simulink model "sschdlexThreePhaseConverterWithGridModel"  (R2026a)
settings: Solver=FixedStepDiscrete  StartTime=0  StopTime=0.09
InitFcn:
  | % LC filter parameters
  | 
  | Lf = 2e-3;
  | Rf = 20e-3;
  | Cf = 1e-6;
  | 
  | % Sample step size
  | 
  | % if ~exist('Tbase')
  |     Tbase = 5e-9;
  | % end
  | 
  | Ts = 1e-6;
  | Tsc=5e-5;
  | fsw = 10e3;
  | 
  | % PWM oversampling
  | oversampling = Ts/Tbase;
  | 
  | % Frame size for data transfer to CPU
  | frame_size = round(Tsc/Ts);
  | 
  | % Control constants
  | 
  | Kp_id = 1.5;
  | Ki_id = 400;
  | Kp_iq = 1.5;
  | Ki_iq = 400;
libraries: simulink x51, hdlsllib x23, fl_lib x15, nesl_utility x15, slrealtimeloglib x12, ee_lib x11, eeTransforms x3, slpidlib x2, eeSinusoidalMeasurement x1
(part 1 of 2)
settings Model: Creator=The MathWorks, Inc.  LastModifiedBy=The MathWorks, Inc.
settings OptimizationCC: ConditionallyExecuteInputs=off
settings DebuggingCC: AlgebraicLoopMsg=error  UnderspecifiedInitializationDetection=Classic  SingleTaskRateTransMsg=error  ParameterPrecisionLossMsg=none
settings HardwareCC: ProdHWDeviceType=ASIC/FPGA->ASIC/FPGA  TargetBitPerLong=64.0  TargetBitPerPointer=64.0  TargetBitPerSizeT=64.0  TargetBitPerPtrDiffT=64.0  TargetLongLongMode=on  TargetIntDivRoundTo=Zero  TargetEndianess=LittleEndian  TargetWordSize=64.0  TargetHWDeviceType=Custom Processor->MATLAB Host Computer  ProdEqTarget=off
settings GRTTargetCC: CombineOutputUpdateFcns=off  GRTInterface=on
settings SimscapeCC: SimscapeNormalizeSystem=off  SimscapeNominalValues="[{\"value\":\"1\",\"unit\":\"A\"},{\"value\":\"1\",\"unit\":\"bar\"},{\"value\":\"1\",\"unit\":\"cm^2\"},{\"value\":\"1\",\"unit\":\"cm^3/s\"},{\"value\":\"1\",\"unit\":\"kJ/kg\"},{\"value\":\"1\",\"unit\":\"kW\"},{\"value\":\"1\",\"unit\":\"l\"},{\"value\":\"1\",\"unit\":\"N\"},{\"value\":\"1\",\"unit\":\"N*m\"},{\"value\":\"1\",\"unit\":\"V\"}]"  SimscapeLogType=none  SimscapeLogDataHistory=5000.0

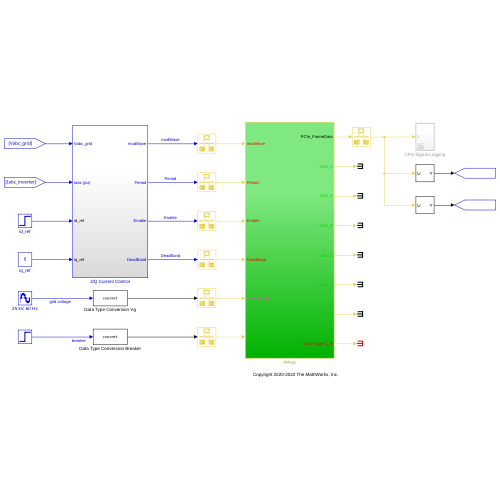
[thumbnail: Simulink's stored preview of the top-level diagram]
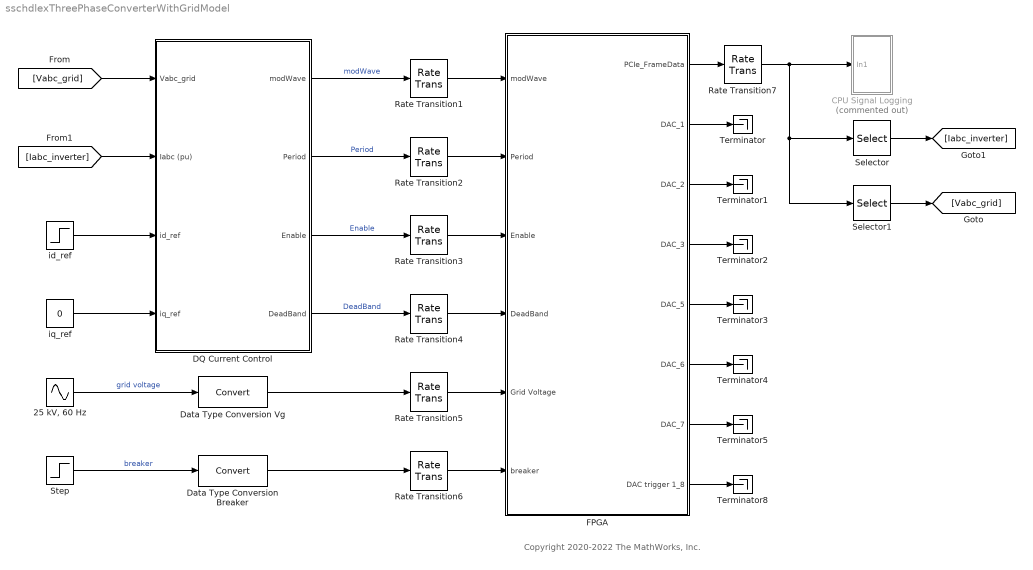
== system sschdlexThreePhaseConverterWithGridModel ==
  note: Copyright 2020-2022 The MathWorks, Inc.
  "25 kV, 60 Hz" : Sin  Amplitude=25000*sqrt(2)/sqrt(3)  Frequency=60*2*pi  Phase=[0 -2*pi/3 2*pi/3]  SampleTime=Tsc
  CPU Signal Logging : Subsystem  Commented=on
  DQ Current Control : Subsystem
  Data Type Conversion Breaker : DataTypeConversion  SaturateOnIntegerOverflow=off  RndMeth=Floor
  Data Type Conversion Vg : DataTypeConversion  SaturateOnIntegerOverflow=off  RndMeth=Floor
  FPGA : Subsystem
  Rate Transition{1..4} (4 alike) : RateTransition  OutPortSampleTime=Tbase
  Rate Transition5 : RateTransition  OutPortSampleTime=Ts
  Rate Transition6 : RateTransition  OutPortSampleTime=Ts
  Rate Transition7 : RateTransition  OutPortSampleTime=Tsc
  Selector : Selector  InputPortWidth=6*frame_size  IndexOptions=Index vector (dialog)  Indices=[1, frame_size+1, 2*frame_size+1]  OutputSizes=1
  Selector1 : Selector  InputPortWidth=6*frame_size  IndexOptions=Index vector (dialog)  Indices=[3*frame_size+1, 4*frame_size+1, 5*frame_size+1]  OutputSizes=1
  Step : Step  Time=0.03  SampleTime=Tsc
  Terminator{,1..5,8} (7 alike) : Terminator
  id_ref : Step  Time=0.06  FinalValue=0.5  SampleTime=Tsc
  iq_ref : Constant  Value=0  SampleTime=Tsc
  wires:
  DQ Current Control/1(modWave) -> Rate Transition1/1  "modWave"
  DQ Current Control/2(Period) -> Rate Transition2/1  "Period"
  DQ Current Control/4(DeadBand) -> Rate Transition4/1  "DeadBand"
  [Iabc_inverter] -> DQ Current Control/2(Iabc (pu))
  [Vabc_grid] -> DQ Current Control/1(Vabc_grid)
  DQ Current Control/3(Enable) -> Rate Transition3/1  "Enable"
  Step/1 -> Data Type Conversion Breaker/1  "breaker"
  FPGA/2(DAC_1) -> Terminator/1
  FPGA/3(DAC_2) -> Terminator1/1
  FPGA/4(DAC_3) -> Terminator2/1
  FPGA/5(DAC_5) -> Terminator3/1
  FPGA/6(DAC_6) -> Terminator4/1
  FPGA/7(DAC_7) -> Terminator5/1
  "25 kV, 60 Hz"/1 -> Data Type Conversion Vg/1  "grid voltage"
  FPGA/8(DAC trigger 1_8) -> Terminator8/1
  Rate Transition1/1 -> FPGA/1(modWave)
  Rate Transition2/1 -> FPGA/2(Period)
  Rate Transition3/1 -> FPGA/3(Enable)
  Rate Transition4/1 -> FPGA/4(DeadBand)
  Rate Transition5/1 -> FPGA/5(Grid Voltage)
  Rate Transition6/1 -> FPGA/6(breaker)
  FPGA/1(PCIe_FrameData) -> Rate Transition7/1
  id_ref/1 -> DQ Current Control/3(id_ref)
  iq_ref/1 -> DQ Current Control/4(iq_ref)
  Rate Transition7/1 -> Selector1/1, Selector/1, CPU Signal Logging/1(In1)
  Data Type Conversion Vg/1 -> Rate Transition5/1
  Data Type Conversion Breaker/1 -> Rate Transition6/1
  Selector/1 -> [Iabc_inverter]
  Selector1/1 -> [Vabc_grid]

== system sschdlexThreePhaseConverterWithGridModel/CPU Signal Logging ==
  In1 : Inport
  Demux : Demux  Outputs=12
  File Log{,1..11} (12 alike) : slrealtimeloglib/File Log  decimation=1
  wires:
  Demux/3 -> File Log2/1
  Demux/2 -> File Log1/1
  Demux/1 -> File Log/1
  In1/1 -> Demux/1
  Demux/5 -> File Log4/1
  Demux/12 -> File Log11/1
  Demux/4 -> File Log3/1
  Demux/9 -> File Log8/1
  Demux/6 -> File Log5/1
  Demux/10 -> File Log9/1
  Demux/11 -> File Log10/1
  Demux/8 -> File Log7/1
  Demux/7 -> File Log6/1

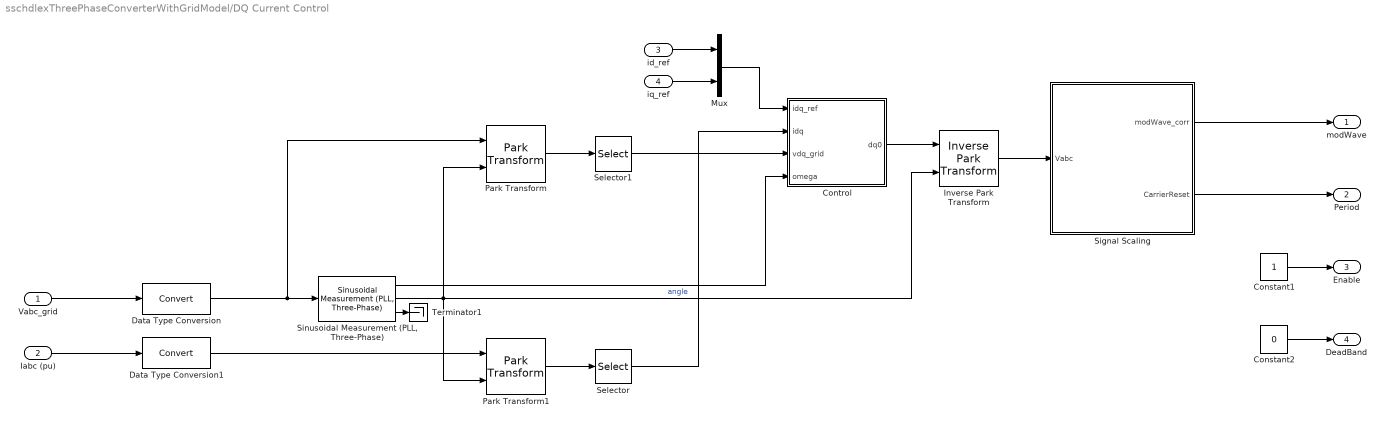
== system sschdlexThreePhaseConverterWithGridModel/DQ Current Control ==
  Vabc_grid : Inport
  Iabc (pu) : Inport  Port=2
  id_ref : Inport  Port=3
  iq_ref : Inport  Port=4
  Constant1 : Constant  OutDataTypeStr=boolean  SampleTime=Tsc
  Constant2 : Constant  Value=0  OutDataTypeStr=uint32  SampleTime=Tsc
  Control : Subsystem
  Data Type Conversion : DataTypeConversion  SaturateOnIntegerOverflow=off  RndMeth=Floor
  Data Type Conversion1 : DataTypeConversion  SaturateOnIntegerOverflow=off  RndMeth=Floor
  Inverse Park Transform : eeTransforms/Inverse Park Transform  AxisAlignment=Q-axis  PowerInvariant=off
  Mux : Mux  Inputs=2
  Park Transform : eeTransforms/Park Transform  AxisAlignment=Q-axis  PowerInvariant=off
  Park Transform1 : eeTransforms/Park Transform  AxisAlignment=Q-axis  PowerInvariant=off
  Selector : Selector  InputPortWidth=3  IndexOptions=Index vector (dialog)  Indices=[1 2]  OutputSizes=1
  Selector1 : Selector  InputPortWidth=3  IndexOptions=Index vector (dialog)  Indices=[1 2]  OutputSizes=1
  Signal Scaling : Subsystem  mask{Vdc=2, fsw=20e3, f_FPGA_clk=1/Tbase}
      mask prompts: fsw "PWM Frequency"; f_FPGA_clk "FPGA Target Frequency"
  "Sinusoidal Measurement (PLL, Three-Phase)" : eeSinusoidalMeasurement/Sinusoidal Measurement (PLL, Three-Phase)  Kp_LF=150  Ki_LF=150  F0=60  Theta0=0  Ts=Tsc
  Terminator1 : Terminator
  modWave : Outport
  Period : Outport  Port=2
  Enable : Outport  Port=3
  DeadBand : Outport  Port=4
  wires:
  Constant1/1 -> Enable/1
  Signal Scaling/1(modWave_corr) -> modWave/1
  Signal Scaling/2(CarrierReset) -> Period/1
  Constant2/1 -> DeadBand/1
  Inverse Park Transform/1 -> Signal Scaling/1(Vabc)
  Mux/1 -> Control/1(idq_ref)
  id_ref/1 -> Mux/1
  iq_ref/1 -> Mux/2
  Selector1/1 -> Control/3(vdq_grid)
  Data Type Conversion/1 -> "Sinusoidal Measurement (PLL, Three-Phase)"/1, Park Transform/1
  "Sinusoidal Measurement (PLL, Three-Phase)"/2 -> Park Transform/2, Inverse Park Transform/2, Park Transform1/2  "angle"
  Control/1(dq0) -> Inverse Park Transform/1
  Park Transform/1 -> Selector1/1
  "Sinusoidal Measurement (PLL, Three-Phase)"/1 -> Control/4(omega)
  Park Transform1/1 -> Selector/1
  Selector/1 -> Control/2(idq)
  "Sinusoidal Measurement (PLL, Three-Phase)"/3 -> Terminator1/1
  Data Type Conversion1/1 -> Park Transform1/1
  Vabc_grid/1 -> Data Type Conversion/1
  Iabc (pu)/1 -> Data Type Conversion1/1

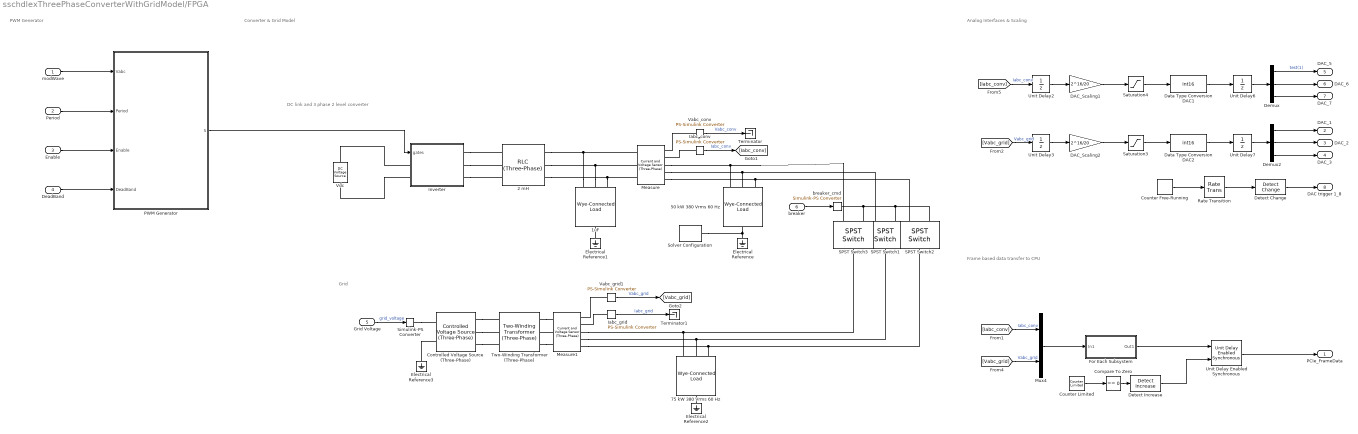
== system sschdlexThreePhaseConverterWithGridModel/FPGA ==
  note: Frame based data transfer to CPU
  note: Analog Interfaces & Scaling
  note: Converter & Grid Model
  note: PWM Generator
  note: Grid
  note: DC link and 3 phase 2 level converter
  modWave : Inport
  Period : Inport  Port=2
  Enable : Inport  Port=3
  DeadBand : Inport  Port=4
  Grid Voltage : Inport  Port=5
  breaker : Inport  Port=6
  1uF : ee_lib/Passive/RLC Assemblies/Wye-Connected Load  port_option=ee.enum.threePhasePort.expanded  parameterization=1  component_structure=3  component_structure_PQ=3  R=1 Ohm  L=0.001 H  C=Cf F  VRated=380 V  FRated=60 Hz  P=0 W  Qpos=0 V*A  Qneg="-54.4375  V*A"  R_parasitic=1e-6 Ohm  G_parasitic=1e-6 1/Ohm  R_parasitic_PQ=1e-6 Ohm  G_parasitic_PQ=1e-6 1/Ohm  Vmag0=380 V  Vang0=0 deg  Freq0=60 Hz  IL_specify=on  IL_priority=High  IL=[ 0 0 0 ] A  IL_nominal_specify=off  IL_nominal_value=1  IL_nominal_unit=A  VC_specify=on  VC_priority=High  VC=[ 0 0 0 ] V  VC_nominal_specify=off  VC_nominal_value=1  VC_nominal_unit=V
  "2 mH " : ee_lib/Passive/RLC Assemblies/RLC (Three-Phase)  port_option=ee.enum.threePhasePort.expanded  component_structure=ee.enum.rlc.structure.SeriesRL  R=Rf Ohm  L=Lf H  C=1 F  R_parasitic=1e-6 Ohm  G_parasitic=1e-6 1/Ohm  IL_specify=on  IL_priority=High  IL=[0, 0, 0] A  IL_nominal_specify=off  IL_nominal_value=1  IL_nominal_unit=A  VC_specify=on  VC_priority=High  VC=[0, 0, 0] V  VC_nominal_specify=off  VC_nominal_value=1  VC_nominal_unit=V
  50 kW 380 Vrms 60 Hz : ee_lib/Passive/RLC Assemblies/Wye-Connected Load  port_option=ee.enum.threePhasePort.expanded  parameterization=2  component_structure=3  component_structure_PQ=1  R=1 Ohm  L=0.001 H  C=1e-6 F  VRated=380 V  FRated=60 Hz  P=50000 W  Qpos=0 V*A  Qneg=-3000 V*A  R_parasitic=1e-6 Ohm  G_parasitic=1e-6 1/Ohm  R_parasitic_PQ=1e-6 Ohm  G_parasitic_PQ=1e-6 1/Ohm  Vmag0=380 V  Vang0=0 deg  Freq0=60 Hz  IL_specify=on  IL_priority=High  IL=[ 0 0 0 ] A  IL_nominal_specify=off  IL_nominal_value=1  IL_nominal_unit=A  VC_specify=on  VC_priority=High  VC=[ 0 0 0 ] V  VC_nominal_specify=off  VC_nominal_value=1  VC_nominal_unit=V
  75 kW 380 Vrms 60 Hz : ee_lib/Passive/RLC Assemblies/Wye-Connected Load  port_option=ee.enum.threePhasePort.expanded  parameterization=2  component_structure=3  component_structure_PQ=1  R=1 Ohm  L=0.001 H  C=1e-6 F  VRated=380 V  FRated=60 Hz  P=75000 W  Qpos=0 V*A  Qneg=-3000 V*A  R_parasitic=1e-6 Ohm  G_parasitic=1e-6 1/Ohm  R_parasitic_PQ=1e-6 Ohm  G_parasitic_PQ=1e-6 1/Ohm  Vmag0=380 V  Vang0=0 deg  Freq0=60 Hz  IL_specify=on  IL_priority=High  IL=[ 0 0 0 ] A  IL_nominal_specify=off  IL_nominal_value=1  IL_nominal_unit=A  VC_specify=on  VC_priority=High  VC=[ 0 0 0 ] V  VC_nominal_specify=off  VC_nominal_value=1  VC_nominal_unit=V
  Compare To Zero : simulink/Logic and Bit Operations/Compare To Zero  relop===  OutDataTypeStr=boolean
  Controlled Voltage Source (Three-Phase) : ee_lib/Sources/Controlled Voltage Source (Three-Phase)  input_option=ee.enum.inputType.instantaneous  FRated=60 Hz
  Counter Free-Running : simulink/Sources/Counter Free-Running  NumBits=1  tsamp=Ts
  Counter Limited : simulink/Sources/Counter Limited  uplimit=frame_size-1  tsamp=Ts
  DAC_Scaling1 : Gain  Gain=2^16/20
  DAC_Scaling2 : Gain  Gain=2^16/20
  Data Type Conversion DAC1 : DataTypeConversion  OutDataTypeStr=int16  SaturateOnIntegerOverflow=off  RndMeth=Floor
  Data Type Conversion DAC2 : DataTypeConversion  OutDataTypeStr=int16  SaturateOnIntegerOverflow=off  RndMeth=Floor
  Demux : Demux  Outputs=3
  Demux2 : Demux  Outputs=3
  Detect Change : simulink/Logic and Bit Operations/Detect Change  vinit=0  OutDataTypeStr=boolean
  Detect Increase : simulink/Logic and Bit Operations/Detect Increase  vinit=0.0  OutDataTypeStr=boolean
  Electrical Reference{,1..3} (4 alike) : fl_lib/Electrical/Electrical Elements/Electrical Reference
  For Each Subsystem : Subsystem  TreatAsAtomicUnit=on
  Iabc_conv : nesl_utility/PS-Simulink Converter  PhysicalDomain=network_engine_domain  SubClassName=ps_output  LeftPortType=input  RightPortType=output  PseudoPeriodic=off  Frequencies=[]  VectorFormat=1-D array  Unit=inherit  AffineConversion=off
  Iabc_grid : nesl_utility/PS-Simulink Converter  PhysicalDomain=network_engine_domain  SubClassName=ps_output  LeftPortType=input  RightPortType=output  PseudoPeriodic=off  Frequencies=[]  VectorFormat=1-D array  Unit=inherit  AffineConversion=off
  Inverter : Subsystem
      mask Display: %image('Inverter.png'); % Use "Edit Image" on toolstrip to change.
  Measure : ee_lib/Sensors & Transducers/Current and Voltage Sensor (Three-Phase)  port_option=ee.enum.threePhasePort.expanded  vMeasurementType=ee.enum.vmeasurement.lg  outputUnit=ee.enum.unit.pu  SRated=150000 V*A  VRated=380 V  I_specify=off  I_priority=None  I=[ 0 0 0 ] A  I_nominal_specify=off  I_nominal_value=1  I_nominal_unit=A  V_specify=off  V_priority=None  V=[ 0 0 0 ] V  V_nominal_specify=off  V_nominal_value=1  V_nominal_unit=V
  Measure1 : ee_lib/Sensors & Transducers/Current and Voltage Sensor (Three-Phase)  port_option=ee.enum.threePhasePort.expanded  vMeasurementType=ee.enum.vmeasurement.lg  outputUnit=ee.enum.unit.pu  SRated=250000 V*A  VRated=380 V  I_specify=off  I_priority=None  I=[ 0 0 0 ] A  I_nominal_specify=off  I_nominal_value=1  I_nominal_unit=A  V_specify=off  V_priority=None  V=[ 0 0 0 ] V  V_nominal_specify=off  V_nominal_value=1  V_nominal_unit=V
  Mux4 : Mux  Inputs=2
  PWM Generator : Subsystem
  Rate Transition : RateTransition  OutPortSampleTime=Tbase
  SPST Switch1 : ee_lib/Switches & Breakers/SPST Switch  R_closed=0.001 Ohm  G_open=1e-6 S  Threshold=0.5 V  Width=0 V  model_dynamics=0  t_on=1e-3 s  t_off=1e-3 s  initial_vT=0 V
  SPST Switch2 : ee_lib/Switches & Breakers/SPST Switch  R_closed=0.001 Ohm  G_open=1e-6 S  Threshold=0.5 V  Width=0 V  model_dynamics=0  t_on=1e-3 s  t_off=1e-3 s  initial_vT=0 V
  SPST Switch3 : ee_lib/Switches & Breakers/SPST Switch  R_closed=0.001 Ohm  G_open=1e-6 S  Threshold=0.5 V  Width=0 V  model_dynamics=0  t_on=1e-3 s  t_off=1e-3 s  initial_vT=0 V
  Saturation3 : Saturate  UpperLimit=2^15-1  LowerLimit=-2^15
  Saturation4 : Saturate  UpperLimit=2^15-1  LowerLimit=-2^15
  Simulink-PS Converter : nesl_utility/Simulink-PS Converter  PhysicalDomain=network_engine_domain  SubClassName=ps_input  LeftPortType=input  RightPortType=output  PseudoPeriodic=off  Frequencies=[]  NoiseDistribution=none  NoiseParameters=[]  Unit=1  AffineConversion=off  FilteringAndDerivatives=provide  SimscapeFilterOrder=1  InputFilterTimeConstant=0.001  UdotUserProvided=0
  Solver Configuration : nesl_utility/Solver Configuration  PhysicalDomain=network_engine_domain  SubClassName=solver  LeftPortType=input  RightPortType=generic  Tones=[]  Harmonics=[]  SimulateNoise=off  Profile=off  UseLocalSampling=off  EnableSwitchedLinearOptims=on  FrequencyDomain=off  UseCCode=off  RelTol=0.001  AbsTol=1e-06  MinStep=1e-09  ToWorkspace=off  RevertToSquareIcSolve=off  NumHomotopyIterations=100  PhasorMode=off  PhasorModeNumHarmonics=1  ConsistencySolver=NEWTON_FTOL  CanonicalOrdering=UNORDERED  OptimizeIntermediates=UNOPTIMIZED  IndexReductionMethod=DerivativeReplacement  DoDC=off  ResidualTolerance=1e-09  ConsistencyTolSource=GLOBAL  ConsistencyAbsTol=0.001  ConsistencyRelTol=0.001  ConsistencyTolFactor=0.001  UseLocalSolver=on  LocalSolverChoice=NE_BACKWARD_EULER_ADVANCER  ResolveIndetEquations=on  FunctionEvalNumThread=1  LocalSolverSampleTime=Ts  DoFixedCost=on  MaxNonlinIter=1  MaxModeIter=2  ComputeImpulses=off  ImpulseIterations=1  LinearAlgebra=Sparse  LinearAlgebraNumThread=0  EquationFormulation=NE_TIME_EF  DelaysMemoryBudget=1024  AutomaticFiltering=on  FilteringTimeConstant=0.001  PartitionStorageMethod=EXHAUSTIVE  PartitionMemoryBudget=1024  PartitionMethod=ROBUST  MultibodyUseLocalSolver=off  MultibodyLocalSolverChoice=ODE1  MultibodyLocalSolverSampleTime=0.001
  Terminator : Terminator
  Terminator1 : Terminator
  Two-Winding Transformer (Three-Phase) : ee_lib/Passive/Transformers/Two-Winding Transformer (Three-Phase)  SRated=500000 V*A  FRated=60 Hz  Winding1Connection=ee.enum.windingconnection.Y  VRated1=25000 V  Winding2Connection=ee.enum.windingconnection.delta1  VRated2=380 V  CoreType=ee.enum.coretype.threelimb  pu_Rw1=0.0020  pu_Rw2=0.0020  leakage_reactance_option=ee.enum.transformer_leakage.include  pu_Xl1=0.0800  pu_Xl2=0.0800  magnetizing_resistance_option=ee.enum.transformer_magnetizingResistance.include  pu_Rm=500  magnetizing_reactance_option=ee.enum.transformer_magnetizingReactance.include  saturation_option=ee.enum.transformer_saturation.exclude  pu_Xm=500  current_data=[0, .002, 1, 2]  magnetic_flux_data=[0, 1.2, 1.5, 1.51]  pu_X0=0.5800  i1_specify=off  i1_priority=None  i1=[ 0 0 0 ] A  i1_nominal_specify=off  i1_nominal_value=1  i1_nominal_unit=A  i2_specify=off  i2_priority=None  i2=[ 0 0 0 ] A  i2_nominal_specify=off  i2_nominal_value=1  i2_nominal_unit=A  phi_specify=off  phi_priority=None  phi=[ 0 0 0 ]  phi_nominal_specify=off  phi_nominal_value=1  phi_nominal_unit=1
  Unit Delay Enabled Synchronous : hdlsllib/Discrete/Unit Delay Enabled Synchronous  InitialCondition=0.0  SampleTime=-1
  Unit Delay{2..3,6..7} (4 alike) : UnitDelay  SampleTime=-1
  Vabc_conv : nesl_utility/PS-Simulink Converter  PhysicalDomain=network_engine_domain  SubClassName=ps_output  LeftPortType=input  RightPortType=output  PseudoPeriodic=off  Frequencies=[]  VectorFormat=1-D array  Unit=inherit  AffineConversion=off
  Vabc_grid1 : nesl_utility/PS-Simulink Converter  PhysicalDomain=network_engine_domain  SubClassName=ps_output  LeftPortType=input  RightPortType=output  PseudoPeriodic=off  Frequencies=[]  VectorFormat=1-D array  Unit=inherit  AffineConversion=off
  Vdc : fl_lib/Electrical/Electrical Sources/DC Voltage Source  v0=1000 V
  breaker_cmd : nesl_utility/Simulink-PS Converter  PhysicalDomain=network_engine_domain  SubClassName=ps_input  LeftPortType=input  RightPortType=output  PseudoPeriodic=off  Frequencies=[]  NoiseDistribution=none  NoiseParameters=[]  Unit=1  AffineConversion=off  FilteringAndDerivatives=provide  SimscapeFilterOrder=1  InputFilterTimeConstant=0.001  UdotUserProvided=0
  PCIe_FrameData : Outport
  DAC_1 : Outport  Port=2
  DAC_2 : Outport  Port=3
  DAC_3 : Outport  Port=4
  DAC_5 : Outport  Port=5
  DAC_6 : Outport  Port=6
  DAC_7 : Outport  Port=7
  DAC trigger 1_8 : Outport  Port=8
  wires:
  DeadBand/1 -> PWM Generator/4(DeadBand)
  modWave/1 -> PWM Generator/1(Vabc)
  Enable/1 -> PWM Generator/3(Enable)
  Period/1 -> PWM Generator/2(Period)
  Counter Free-Running/1 -> Rate Transition/1
  Rate Transition/1 -> Detect Change/1
  Demux/1 -> DAC_5/1  "test(1)"
  Demux/2 -> DAC_6/1
  Demux/3 -> DAC_7/1
  Demux2/1 -> DAC_1/1
  Demux2/2 -> DAC_2/1
  Demux2/3 -> DAC_3/1
  Unit Delay2/1 -> DAC_Scaling1/1
  Unit Delay3/1 -> DAC_Scaling2/1
  DAC_Scaling1/1 -> Saturation4/1
  DAC_Scaling2/1 -> Saturation3/1
  Saturation4/1 -> Data Type Conversion DAC1/1
  Saturation3/1 -> Data Type Conversion DAC2/1
  Unit Delay6/1 -> Demux/1
  Unit Delay7/1 -> Demux2/1
  Data Type Conversion DAC1/1 -> Unit Delay6/1
  Data Type Conversion DAC2/1 -> Unit Delay7/1
  Detect Change/1 -> DAC trigger 1_8/1
  Mux4/1 -> For Each Subsystem/1(In1)
  Iabc_conv/1 -> [Iabc_conv]  "Iabc_conv"
  Vabc_conv/1 -> Terminator/1  "Vabc_conv"
  Vabc_grid1/1 -> [Vabc_grid]  "Vabc_grid"
  Iabc_grid/1 -> Terminator1/1  "Iabc_grid"
  PWM Generator/1(S) -> Inverter/1(gates)
  Grid Voltage/1 -> Simulink-PS Converter/1  "grid_voltage"
  breaker/1 -> breaker_cmd/1
  [Vabc_grid] -> Unit Delay3/1  "Vabc_grid"
  [Iabc_conv] -> Unit Delay2/1  "Iabc_conv"
  [Vabc_grid] -> Mux4/2  "Vabc_grid"
  [Iabc_conv] -> Mux4/1  "Iabc_conv"
  Counter Limited/1 -> Compare To Zero/1
  Compare To Zero/1 -> Detect Increase/1
  Detect Increase/1 -> Unit Delay Enabled Synchronous/2
  Unit Delay Enabled Synchronous/1 -> PCIe_FrameData/1
  For Each Subsystem/1(Out1) -> Unit Delay Enabled Synchronous/1
  connections:
  SPST Switch1/LConn1 -- SPST Switch2/LConn1 -- SPST Switch3/LConn1 -- breaker_cmd/RConn1
  50 kW 380 Vrms 60 Hz/RConn1 -- Electrical Reference/LConn1 -- Solver Configuration/RConn1
  SPST Switch3/RConn1 -- 75 kW 380 Vrms 60 Hz/LConn1 -- Measure1/RConn3
  SPST Switch2/LConn2 -- 50 kW 380 Vrms 60 Hz/LConn3 -- Measure/RConn5
  50 kW 380 Vrms 60 Hz/LConn1 -- SPST Switch3/LConn2 -- Measure/RConn3
  1uF/LConn1 -- Measure/LConn1 -- "2 mH "/RConn1
  SPST Switch2/RConn1 -- 75 kW 380 Vrms 60 Hz/LConn3 -- Measure1/RConn5
  1uF/LConn3 -- Measure/LConn3 -- "2 mH "/RConn3
  SPST Switch1/LConn2 -- 50 kW 380 Vrms 60 Hz/LConn2 -- Measure/RConn4
  1uF/LConn2 -- Measure/LConn2 -- "2 mH "/RConn2
  SPST Switch1/RConn1 -- 75 kW 380 Vrms 60 Hz/LConn2 -- Measure1/RConn4
  Electrical Reference3/LConn1 -- Controlled Voltage Source (Three-Phase)/LConn2
  Inverter/RConn3 -- "2 mH "/LConn3
  Controlled Voltage Source (Three-Phase)/RConn3 -- Two-Winding Transformer (Three-Phase)/LConn3
  Controlled Voltage Source (Three-Phase)/RConn1 -- Two-Winding Transformer (Three-Phase)/LConn1
  Measure1/LConn2 -- Two-Winding Transformer (Three-Phase)/RConn2
  Iabc_conv/LConn1 -- Measure/RConn2
  Iabc_grid/LConn1 -- Measure1/RConn2
  Inverter/LConn1 -- Vdc/LConn1
  Inverter/RConn2 -- "2 mH "/LConn2
  Simulink-PS Converter/RConn1 -- Controlled Voltage Source (Three-Phase)/LConn1
  Two-Winding Transformer (Three-Phase)/RConn3 -- Measure1/LConn3
  Vabc_conv/LConn1 -- Measure/RConn1
  Electrical Reference2/LConn1 -- 75 kW 380 Vrms 60 Hz/RConn1
  Controlled Voltage Source (Three-Phase)/RConn2 -- Two-Winding Transformer (Three-Phase)/LConn2
  Two-Winding Transformer (Three-Phase)/RConn1 -- Measure1/LConn1
  Inverter/RConn1 -- "2 mH "/LConn1
  Vabc_grid1/LConn1 -- Measure1/RConn1
  Inverter/LConn2 -- Vdc/RConn1
  Electrical Reference1/LConn1 -- 1uF/RConn1

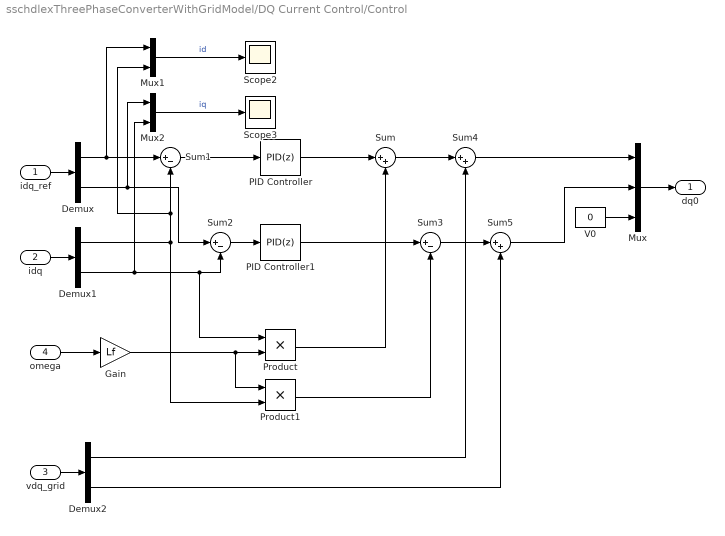
== system sschdlexThreePhaseConverterWithGridModel/DQ Current Control/Control ==
  idq_ref : Inport
  idq : Inport  Port=2
  vdq_grid : Inport  Port=3
  omega : Inport  Port=4
  Demux : Demux  Outputs=2
  Demux1 : Demux  Outputs=2
  Demux2 : Demux  Outputs=2
  Gain : Gain  Gain=Lf
  Mux : Mux  Inputs=3
  Mux1 : Mux  Inputs=2
  Mux2 : Mux  Inputs=2
  PID Controller : slpidlib/PID Controller  Controller=PID  Form=Parallel  TimeDomain=Discrete-time  UseExternalTs=off  SampleTime=-1  IntegratorMethod=Forward Euler  FilterMethod=Forward Euler  ControllerParametersSource=internal  P=Kp_id  I=Ki_id  UseKiTs=off  D=0  UseExternalDerivativeSource=off  N=100  UseFilter=off  TunerSelectOption=Transfer Function Based (PID Tuner App)  InitialConditionSource=internal  InitialConditionForIntegrator=0  InitialConditionForFilter=0  DifferentiatorICPrevScaledInput=0  ExternalReset=none  TrackingMode=off  Kt=1  LimitOutput=on  SatLimitsSource=internal  UpperSaturationLimit=3  LowerSaturationLimit=-3  LinearizeAsGain=on  AntiWindupMode=back-calculation  Kb=100  LimitIntegrator=off  UpperIntegratorSaturationLimit=inf  LowerIntegratorSaturationLimit=-inf  POutMin=[]  POutMax=[]  IOutMin=[]  IOutMax=[]  DOutMin=[]  DOutMax=[]  NOutMin=[]  NOutMax=[]  SumOutMin=[]  SumOutMax=[]  SaturationOutMin=[]  SaturationOutMax=[]  PParamMin=[]  PParamMax=[]  IParamMin=[]  IParamMax=[]  DParamMin=[]  DParamMax=[]  NParamMin=[]  NParamMax=[]  KbParamMin=[]  KbParamMax=[]  KtParamMin=[]  KtParamMax=[]  KbOutMin=[]  KbOutMax=[]  KtOutMin=[]  KtOutMax=[]  IntegratorOutMin=[]  IntegratorOutMax=[]  FilterOutMin=[]  FilterOutMax=[]  SumI1OutMin=[]  SumI1OutMax=[]  SumI2OutMin=[]  SumI2OutMax=[]  SumI3OutMin=[]  SumI3OutMax=[]  SumI4OutMin=[]  SumI4OutMax=[]  SumDOutMin=[]  SumDOutMax=[]  DifferentiatorOutMin=[]  DifferentiatorOutMax=[]  FilterDiffOutCoefMin=[]  FilterDiffOutCoefMax=[]  ReciprocalOutMin=[]  ReciprocalOutMax=[]  SumDenOutMin=[]  SumDenOutMax=[]  SumNumOutMin=[]  SumNumOutMax=[]  DivideOutMin=[]  DivideOutMax=[]  UdiffTsProdOutMin=[]  UdiffTsProdOutMax=[]  NTsProdOutMin=[]  NTsProdOutMax=[]  UintegralTsProdOutMin=[]  UintegralTsProdOutMax=[]  UngainTsProdOutMin=[]  UngainTsProdOutMax=[]  ClampingZeroOutDataTypeStr=Inherit: Inherit via back propagation  ClampingZeroOutMin=[]  ClampingZeroOutMax=[]  FilterDenConstantOutDataTypeStr=Inherit: Inherit via back propagation  FilterDenConstantOutMin=[]  FilterDenConstantOutMax=[]  PCopyOutDataTypeStr=Inherit: Inherit via back propagation  PCopyOutMin=[]  PCopyOutMax=[]  NCopyOutDataTypeStr=Inherit: Inherit via back propagation  NCopyOutMin=[]  NCopyOutMax=[]  IntegratorContinuousStateAttributes=''  IntegratorStateMustResolveToSignalObject=off  IntegratorRTWStateStorageClass=Auto  FilterContinuousStateAttributes=''  FilterStateMustResolveToSignalObject=off  FilterRTWStateStorageClass=Auto  ParallelPVariant=InternalParameters  IdealPVariant=Disabled  IVariant=InternalParameters  DVariant=InternalParameters  IntegratorVariant=Discrete  SatVariant=Enabled  AWVariant=BackCalculation  PCopyVariant=Disabled  TRVariant=Disabled  FdbkBlocksVariant=Forward  IdealPFdbkVariant=Disabled  SatFdbkVariant=Disabled  DerivativeFilterVariant=Differentiator  NVariant=Passthrough  NCopyVariant=Disabled_SignalSpec  FilterICVariant=InternalICsDifferentiator  IntegratorICVariant=InternalICs  ExternalResetVariant=Disabled  TRSumVariant=Passthrough  SumFdbkVariant=Disabled  SumVariant=Sum_PID  TsampFilterVariant=InternalTs  TsampNgainVariant=Passthrough  TsampIntegralVariant=Disabled_SignalSpec  ExternalSaturationOutDataTypeStr=Inherit: Same as second input  DerivativeSourceVariant=ErrorSignal  PreIntVariant=InternalPreInt
  PID Controller1 : slpidlib/PID Controller  Controller=PID  Form=Parallel  TimeDomain=Discrete-time  UseExternalTs=off  SampleTime=-1  IntegratorMethod=Forward Euler  FilterMethod=Forward Euler  ControllerParametersSource=internal  P=Kp_iq  I=Ki_iq  UseKiTs=off  D=0  UseExternalDerivativeSource=off  N=100  UseFilter=off  TunerSelectOption=Transfer Function Based (PID Tuner App)  InitialConditionSource=internal  InitialConditionForIntegrator=0  InitialConditionForFilter=0  DifferentiatorICPrevScaledInput=0  ExternalReset=none  TrackingMode=off  Kt=1  LimitOutput=on  SatLimitsSource=internal  UpperSaturationLimit=3  LowerSaturationLimit=-3  LinearizeAsGain=on  AntiWindupMode=back-calculation  Kb=100  LimitIntegrator=off  UpperIntegratorSaturationLimit=inf  LowerIntegratorSaturationLimit=-inf  POutMin=[]  POutMax=[]  IOutMin=[]  IOutMax=[]  DOutMin=[]  DOutMax=[]  NOutMin=[]  NOutMax=[]  SumOutMin=[]  SumOutMax=[]  SaturationOutMin=[]  SaturationOutMax=[]  PParamMin=[]  PParamMax=[]  IParamMin=[]  IParamMax=[]  DParamMin=[]  DParamMax=[]  NParamMin=[]  NParamMax=[]  KbParamMin=[]  KbParamMax=[]  KtParamMin=[]  KtParamMax=[]  KbOutMin=[]  KbOutMax=[]  KtOutMin=[]  KtOutMax=[]  IntegratorOutMin=[]  IntegratorOutMax=[]  FilterOutMin=[]  FilterOutMax=[]  SumI1OutMin=[]  SumI1OutMax=[]  SumI2OutMin=[]  SumI2OutMax=[]  SumI3OutMin=[]  SumI3OutMax=[]  SumI4OutMin=[]  SumI4OutMax=[]  SumDOutMin=[]  SumDOutMax=[]  DifferentiatorOutMin=[]  DifferentiatorOutMax=[]  FilterDiffOutCoefMin=[]  FilterDiffOutCoefMax=[]  ReciprocalOutMin=[]  ReciprocalOutMax=[]  SumDenOutMin=[]  SumDenOutMax=[]  SumNumOutMin=[]  SumNumOutMax=[]  DivideOutMin=[]  DivideOutMax=[]  UdiffTsProdOutMin=[]  UdiffTsProdOutMax=[]  NTsProdOutMin=[]  NTsProdOutMax=[]  UintegralTsProdOutMin=[]  UintegralTsProdOutMax=[]  UngainTsProdOutMin=[]  UngainTsProdOutMax=[]  ClampingZeroOutDataTypeStr=Inherit: Inherit via back propagation  ClampingZeroOutMin=[]  ClampingZeroOutMax=[]  FilterDenConstantOutDataTypeStr=Inherit: Inherit via back propagation  FilterDenConstantOutMin=[]  FilterDenConstantOutMax=[]  PCopyOutDataTypeStr=Inherit: Inherit via back propagation  PCopyOutMin=[]  PCopyOutMax=[]  NCopyOutDataTypeStr=Inherit: Inherit via back propagation  NCopyOutMin=[]  NCopyOutMax=[]  IntegratorContinuousStateAttributes=''  IntegratorStateMustResolveToSignalObject=off  IntegratorRTWStateStorageClass=Auto  FilterContinuousStateAttributes=''  FilterStateMustResolveToSignalObject=off  FilterRTWStateStorageClass=Auto  ParallelPVariant=InternalParameters  IdealPVariant=Disabled  IVariant=InternalParameters  DVariant=InternalParameters  IntegratorVariant=Discrete  SatVariant=Enabled  AWVariant=BackCalculation  PCopyVariant=Disabled  TRVariant=Disabled  FdbkBlocksVariant=Forward  IdealPFdbkVariant=Disabled  SatFdbkVariant=Disabled  DerivativeFilterVariant=Differentiator  NVariant=Passthrough  NCopyVariant=Disabled_SignalSpec  FilterICVariant=InternalICsDifferentiator  IntegratorICVariant=InternalICs  ExternalResetVariant=Disabled  TRSumVariant=Passthrough  SumFdbkVariant=Disabled  SumVariant=Sum_PID  TsampFilterVariant=InternalTs  TsampNgainVariant=Passthrough  TsampIntegralVariant=Disabled_SignalSpec  ExternalSaturationOutDataTypeStr=Inherit: Same as second input  DerivativeSourceVariant=ErrorSignal  PreIntVariant=InternalPreInt
  Product : Product
  Product1 : Product
  Scope2 : Scope
      settings: ActiveDisplayYMinimum=-1.23441  ActiveDisplayYMaximum=0.69271  DataLoggingVariableName=id
  Scope3 : Scope
      settings: ActiveDisplayYMinimum=-0.35108  ActiveDisplayYMaximum=0.28909  DataLoggingVariableName=iq
  Sum : Sum  Inputs=|++
  Sum1 : Sum  Inputs=|+-
  Sum2 : Sum  Inputs=|+-
  Sum3 : Sum  Inputs=|+-
  Sum4 : Sum  Inputs=|++
  Sum5 : Sum  Inputs=|++
  V0 : Constant  Value=0  SampleTime=-1
  dq0 : Outport
  wires:
  Mux/1 -> dq0/1
  idq_ref/1 -> Demux/1
  idq/1 -> Demux1/1
  Demux/1 -> Mux1/1, Sum1/1
  Demux/2 -> Sum2/1, Mux2/1
  Demux1/2 -> Product/1, Sum2/2, Mux2/2
  Sum1/1 -> PID Controller/1
  Sum2/1 -> PID Controller1/1
  PID Controller/1 -> Sum/1
  Product/1 -> Sum/2
  omega/1 -> Gain/1
  Gain/1 -> Product1/1, Product/2
  PID Controller1/1 -> Sum3/1
  Product1/1 -> Sum3/2
  Demux1/1 -> Product1/2, Mux1/2, Sum1/2
  Sum/1 -> Sum4/1
  Sum3/1 -> Sum5/1
  vdq_grid/1 -> Demux2/1
  Demux2/1 -> Sum4/2
  Demux2/2 -> Sum5/2
  Sum4/1 -> Mux/1
  Sum5/1 -> Mux/2
  V0/1 -> Mux/3
  Mux1/1 -> Scope2/1  "id"
  Mux2/1 -> Scope3/1  "iq"

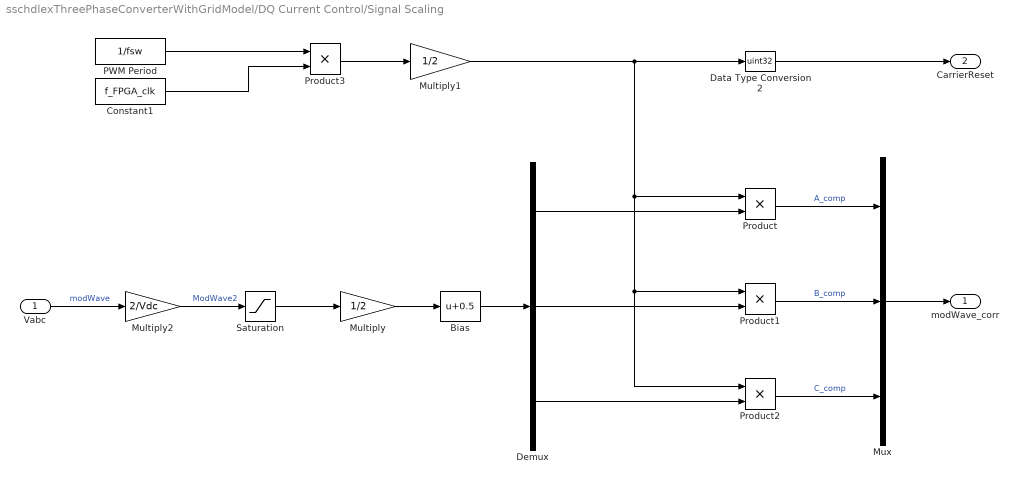
== system sschdlexThreePhaseConverterWithGridModel/DQ Current Control/Signal Scaling ==
  Vabc : Inport
  Bias : Bias  Bias=0.5  SaturateOnIntegerOverflow=off
  Constant1 : Constant  Value=f_FPGA_clk  SampleTime=-1
  Data Type Conversion2 : DataTypeConversion  OutDataTypeStr=uint32  SaturateOnIntegerOverflow=off  RndMeth=Floor
  Demux : Demux  Outputs=3
  Multiply : Gain  Gain=1/2
  Multiply1 : Gain  Gain=1/2
  Multiply2 : Gain  Gain=2/Vdc
  Mux : Mux  Inputs=3
  PWM Period : Constant  Value=1/fsw  SampleTime=-1
  Product : Product  OutDataTypeStr=uint32
  Product1 : Product  OutDataTypeStr=uint32
  Product2 : Product  OutDataTypeStr=uint32
  Product3 : Product
  Saturation : Saturate  UpperLimit=1  LowerLimit=-1
  modWave_corr : Outport  VectorParamsAs1DForOutWhenUnconnected=off
  CarrierReset : Outport  Port=2  VectorParamsAs1DForOutWhenUnconnected=off
  wires:
  Vabc/1 -> Multiply2/1  "modWave"
  Multiply1/1 -> Data Type Conversion2/1, Product/1, Product2/1, Product1/1
  PWM Period/1 -> Product3/1
  Data Type Conversion2/1 -> CarrierReset/1
  Demux/1 -> Product/2
  Demux/2 -> Product1/2
  Demux/3 -> Product2/2
  Constant1/1 -> Product3/2
  Product3/1 -> Multiply1/1
  Product1/1 -> Mux/2  "B_comp"
  Product/1 -> Mux/1  "A_comp"
  Product2/1 -> Mux/3  "C_comp"
  Bias/1 -> Demux/1
  Multiply/1 -> Bias/1
  Mux/1 -> modWave_corr/1
  Multiply2/1 -> Saturation/1  "ModWave2"
  Saturation/1 -> Multiply/1

== system sschdlexThreePhaseConverterWithGridModel/FPGA/For Each Subsystem ==
  In1 : Inport  Partition=on  PartitionDimension=1  PartitionWidth=1  PartitionOffset=0
  For Each : ForEach  DisableCoverage=on
  Tapped Delay : simulink/Discrete/Tapped Delay  vinit=0.0  samptime=Ts  NumDelays=frame_size  DelayOrder=Oldest  includeCurrent=off
  Out1 : Outport  ConcatenationDimension=1
  wires:
  In1/1 -> Tapped Delay/1
  Tapped Delay/1 -> Out1/1

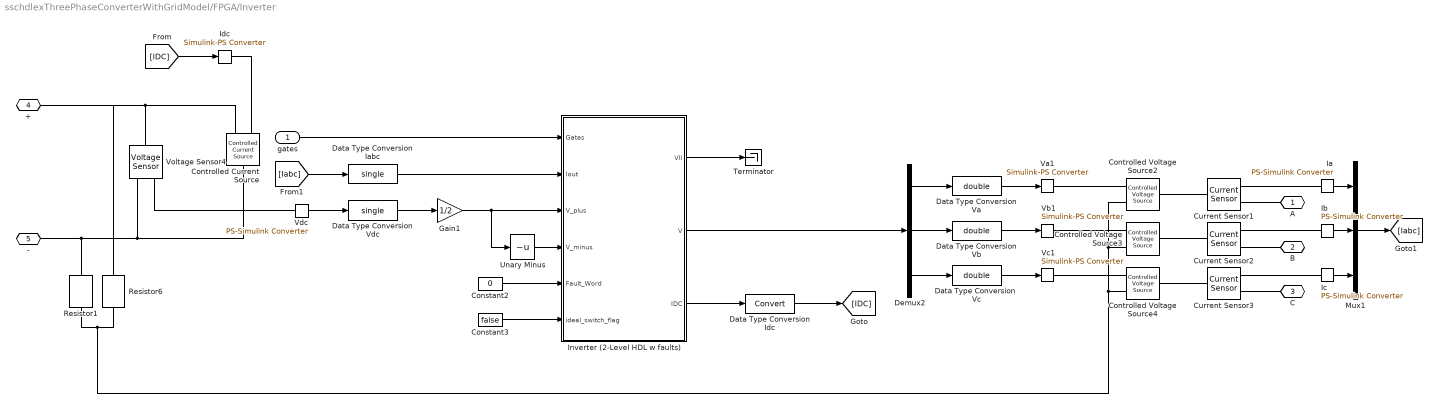
== system sschdlexThreePhaseConverterWithGridModel/FPGA/Inverter ==
  gates : Inport
  Constant2 : Constant  Value=0  OutDataTypeStr=uint32  SampleTime=-1
  Constant3 : Constant  Value=false  SampleTime=-1
  Controlled Current Source : fl_lib/Electrical/Electrical Sources/Controlled Current Source
  Controlled Voltage Source2 : fl_lib/Electrical/Electrical Sources/Controlled Voltage Source
  Controlled Voltage Source3 : fl_lib/Electrical/Electrical Sources/Controlled Voltage Source
  Controlled Voltage Source4 : fl_lib/Electrical/Electrical Sources/Controlled Voltage Source
  Current Sensor1 : fl_lib/Electrical/Electrical Sensors/Current Sensor
  Current Sensor2 : fl_lib/Electrical/Electrical Sensors/Current Sensor
  Current Sensor3 : fl_lib/Electrical/Electrical Sensors/Current Sensor
  Data Type Conversion  Vc : DataTypeConversion  OutDataTypeStr=double  RndMeth=Nearest  SaturateOnIntegerOverflow=off
  Data Type Conversion Iabc : DataTypeConversion  OutDataTypeStr=single  RndMeth=Nearest  SaturateOnIntegerOverflow=off
  Data Type Conversion Idc : DataTypeConversion  RndMeth=Nearest  SaturateOnIntegerOverflow=off
  Data Type Conversion Va : DataTypeConversion  OutDataTypeStr=double  RndMeth=Nearest  SaturateOnIntegerOverflow=off
  Data Type Conversion Vb : DataTypeConversion  OutDataTypeStr=double  RndMeth=Nearest  SaturateOnIntegerOverflow=off
  Data Type Conversion Vdc : DataTypeConversion  OutDataTypeStr=single  RndMeth=Nearest  SaturateOnIntegerOverflow=off
  Demux2 : Demux  Outputs=3
  Gain1 : Gain  Gain=1/2
  Ia : nesl_utility/PS-Simulink Converter  PhysicalDomain=network_engine_domain  SubClassName=ps_output  LeftPortType=input  RightPortType=output  PseudoPeriodic=off  Frequencies=[]  VectorFormat=1-D array  Unit=inherit  AffineConversion=off
  Ib : nesl_utility/PS-Simulink Converter  PhysicalDomain=network_engine_domain  SubClassName=ps_output  LeftPortType=input  RightPortType=output  PseudoPeriodic=off  Frequencies=[]  VectorFormat=1-D array  Unit=inherit  AffineConversion=off
  Ic : nesl_utility/PS-Simulink Converter  PhysicalDomain=network_engine_domain  SubClassName=ps_output  LeftPortType=input  RightPortType=output  PseudoPeriodic=off  Frequencies=[]  VectorFormat=1-D array  Unit=inherit  AffineConversion=off
  Idc : nesl_utility/Simulink-PS Converter  PhysicalDomain=network_engine_domain  SubClassName=ps_input  LeftPortType=input  RightPortType=output  PseudoPeriodic=off  Frequencies=[]  NoiseDistribution=none  NoiseParameters=[]  Unit=1  AffineConversion=off  FilteringAndDerivatives=provide  SimscapeFilterOrder=1  InputFilterTimeConstant=0.001  UdotUserProvided=0
  Inverter (2-Level HDL w faults) : Subsystem  mask{rSnub=10000, rSwitch=0.001, vfSwitch=0, rDiode=0.001, vfDiode=0.8, ts_FPGA_clk=Tbase, ts_FPGA_mdl=Ts}
      mask prompts: rSnub "Snubber Resistance (Ohms)"; rSwitch "Switch Resistance (Ohms)"; vfSwitch "Switch Forward Voltage (V)"; rDiode "Diode Resistance (Ohms)"; vfDiode "Diode Forward Voltage (V)"; ts_FPGA_clk "FPGA clock tick (s)"; ts_FPGA_mdl "Model sample step (s)"
  Mux1 : Mux  Inputs=3
  Resistor1 : fl_lib/Electrical/Electrical Elements/Resistor  R=10000 Ohm  i_specify=off  i_priority=None  i=0 A  i_nominal_specify=off  i_nominal_value=1  i_nominal_unit=A  v_specify=off  v_priority=None  v=0 V  v_nominal_specify=off  v_nominal_value=1  v_nominal_unit=V
  Resistor6 : fl_lib/Electrical/Electrical Elements/Resistor  R=10000 Ohm  i_specify=off  i_priority=None  i=0 A  i_nominal_specify=off  i_nominal_value=1  i_nominal_unit=A  v_specify=off  v_priority=None  v=0 V  v_nominal_specify=off  v_nominal_value=1  v_nominal_unit=V
  Terminator : Terminator
  Unary Minus : UnaryMinus
  Va1 : nesl_utility/Simulink-PS Converter  PhysicalDomain=network_engine_domain  SubClassName=ps_input  LeftPortType=input  RightPortType=output  PseudoPeriodic=off  Frequencies=[]  NoiseDistribution=none  NoiseParameters=[]  Unit=1  AffineConversion=off  FilteringAndDerivatives=provide  SimscapeFilterOrder=1  InputFilterTimeConstant=0.001  UdotUserProvided=0
  Vb1 : nesl_utility/Simulink-PS Converter  PhysicalDomain=network_engine_domain  SubClassName=ps_input  LeftPortType=input  RightPortType=output  PseudoPeriodic=off  Frequencies=[]  NoiseDistribution=none  NoiseParameters=[]  Unit=1  AffineConversion=off  FilteringAndDerivatives=provide  SimscapeFilterOrder=1  InputFilterTimeConstant=0.001  UdotUserProvided=0
  Vc1 : nesl_utility/Simulink-PS Converter  PhysicalDomain=network_engine_domain  SubClassName=ps_input  LeftPortType=input  RightPortType=output  PseudoPeriodic=off  Frequencies=[]  NoiseDistribution=none  NoiseParameters=[]  Unit=1  AffineConversion=off  FilteringAndDerivatives=provide  SimscapeFilterOrder=1  InputFilterTimeConstant=0.001  UdotUserProvided=0
  Vdc : nesl_utility/PS-Simulink Converter  PhysicalDomain=network_engine_domain  SubClassName=ps_output  LeftPortType=input  RightPortType=output  PseudoPeriodic=off  Frequencies=[]  VectorFormat=1-D array  Unit=inherit  AffineConversion=off
  Voltage Sensor4 : fl_lib/Electrical/Electrical Sensors/Voltage Sensor
  A : PMIOPort  Side=Right
  B : PMIOPort  Port=2  Side=Right
  C : PMIOPort  Port=3  Side=Right
  + : PMIOPort  Port=4  Side=Left
  - : PMIOPort  Port=5  Side=Left
  wires:
  Vdc/1 -> Data Type Conversion Vdc/1
  Unary Minus/1 -> Inverter (2-Level HDL w faults)/4(V_minus)
  Data Type Conversion Idc/1 -> [IDC]
  gates/1 -> Inverter (2-Level HDL w faults)/1(Gates)
  Constant3/1 -> Inverter (2-Level HDL w faults)/6(ideal_switch_flag)
  Data Type Conversion Iabc/1 -> Inverter (2-Level HDL w faults)/2(Iout)
  Data Type Conversion Vdc/1 -> Gain1/1
  Inverter (2-Level HDL w faults)/1(Vll) -> Terminator/1
  Constant2/1 -> Inverter (2-Level HDL w faults)/5(Fault_Word)
  Inverter (2-Level HDL w faults)/3(IDC) -> Data Type Conversion Idc/1
  [Iabc] -> Data Type Conversion Iabc/1
  [IDC] -> Idc/1
  Ib/1 -> Mux1/2
  Ic/1 -> Mux1/3
  Ia/1 -> Mux1/1
  Mux1/1 -> [Iabc]
  Inverter (2-Level HDL w faults)/2(V) -> Demux2/1
  Demux2/2 -> Data Type Conversion Vb/1
  Data Type Conversion Va/1 -> Va1/1
  Demux2/3 -> Data Type Conversion  Vc/1
  Demux2/1 -> Data Type Conversion Va/1
  Data Type Conversion Vb/1 -> Vb1/1
  Data Type Conversion  Vc/1 -> Vc1/1
  Gain1/1 -> Inverter (2-Level HDL w faults)/3(V_plus), Unary Minus/1
  connections:
  -/RConn1 -- Controlled Current Source/LConn1 -- Voltage Sensor4/RConn2 -- Resistor1/RConn1
  Voltage Sensor4/LConn1 -- Controlled Current Source/RConn2 -- +/RConn1 -- Resistor6/LConn1
  Idc/RConn1 -- Controlled Current Source/RConn1
  Voltage Sensor4/RConn1 -- Vdc/LConn1
  Current Sensor3/RConn1 -- Ic/LConn1
  Current Sensor1/RConn1 -- Ia/LConn1
  Ib/LConn1 -- Current Sensor2/RConn1
  Current Sensor1/RConn2 -- A/RConn1
  Current Sensor2/RConn2 -- B/RConn1
  Current Sensor3/RConn2 -- C/RConn1
  Va1/RConn1 -- Controlled Voltage Source2/RConn1
  Vb1/RConn1 -- Controlled Voltage Source3/RConn1
  Vc1/RConn1 -- Controlled Voltage Source4/RConn1
  Controlled Voltage Source4/LConn1 -- Current Sensor3/LConn1
  Controlled Voltage Source3/LConn1 -- Current Sensor2/LConn1
  Controlled Voltage Source2/LConn1 -- Current Sensor1/LConn1
  Controlled Voltage Source2/RConn2 -- Controlled Voltage Source4/RConn2 -- Resistor1/LConn1 -- Resistor6/RConn1 -- Controlled Voltage Source3/RConn2

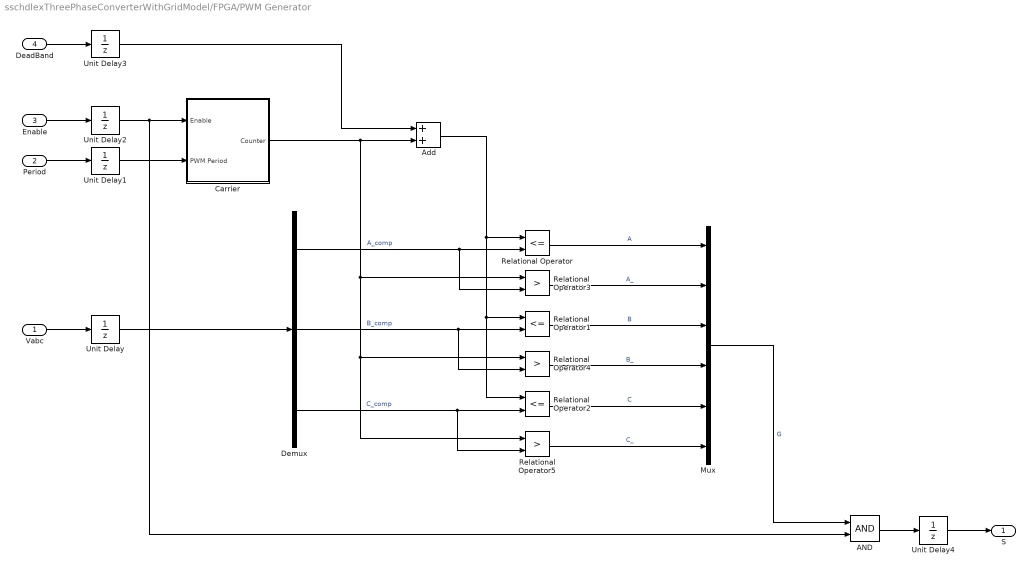
== system sschdlexThreePhaseConverterWithGridModel/FPGA/PWM Generator ==
  Vabc : Inport
  Period : Inport  Port=2
  Enable : Inport  Port=3
  DeadBand : Inport  Port=4
  AND : Logic  AllPortsSameDT=off  OutDataTypeStr=boolean
  Add : Sum
  Carrier : Subsystem
  Demux : Demux  Outputs=3
  Mux : Mux  Inputs=6
  Relational Operator : RelationalOperator  Operator=<=  OutDataTypeStr=boolean  InputSameDT=off
  Relational Operator1 : RelationalOperator  Operator=<=  OutDataTypeStr=boolean  InputSameDT=off
  Relational Operator2 : RelationalOperator  Operator=<=  OutDataTypeStr=boolean  InputSameDT=off
  Relational Operator3 : RelationalOperator  Operator=>  OutDataTypeStr=boolean  InputSameDT=off
  Relational Operator4 : RelationalOperator  Operator=>  OutDataTypeStr=boolean  InputSameDT=off
  Relational Operator5 : RelationalOperator  Operator=>  OutDataTypeStr=boolean  InputSameDT=off
  Unit Delay{,1..4} (5 alike) : UnitDelay  SampleTime=-1
  S : Outport  VectorParamsAs1DForOutWhenUnconnected=off
  wires:
  Period/1 -> Unit Delay1/1
  Mux/1 -> AND/1  "G"
  Enable/1 -> Unit Delay2/1
  Relational Operator5/1 -> Mux/6  "C_"
  Relational Operator2/1 -> Mux/5  "C"
  Relational Operator3/1 -> Mux/2  "A_"
  Vabc/1 -> Unit Delay/1
  Relational Operator4/1 -> Mux/4  "B_"
  Relational Operator/1 -> Mux/1  "A"
  Relational Operator1/1 -> Mux/3  "B"
  Demux/1 -> Relational Operator3/2, Relational Operator/2  "A_comp"
  Demux/2 -> Relational Operator4/2, Relational Operator1/2  "B_comp"
  Demux/3 -> Relational Operator5/2, Relational Operator2/2  "C_comp"
  Carrier/1(Counter) -> Add/2, Relational Operator3/1, Relational Operator4/1, Relational Operator5/1
  DeadBand/1 -> Unit Delay3/1
  Add/1 -> Relational Operator2/1, Relational Operator1/1, Relational Operator/1
  Unit Delay/1 -> Demux/1
  Unit Delay1/1 -> Carrier/2(PWM Period)
  Unit Delay2/1 -> AND/2, Carrier/1(Enable)
  Unit Delay3/1 -> Add/1
  Unit Delay4/1 -> S/1
  AND/1 -> Unit Delay4/1
